simulink model "model"  (R2024a)
settings: Solver=FixedStepDiscrete  StartTime=0.0  StopTime=Tend  FixedStep=Ts  RelTol=1e-3
PreLoadFcn:
  | release_bus_types;
InitFcn:
  | release_initialize(p1,p2,p3,p4);
StartFcn:
  | % MG_4bus_ini;
values from neighbouring files (symbols this model uses):
  dPQload_max = 100*S_b    (= 100000)    [ini.m]
  f_b = 60    [ini.m]
  I_b = S_b/(sqrt(3)*V_b)    [ini.m]
  S_b = 1e3    (= 1000)    [ini.m]
  V_b = 230    [ini.m]
  V_m = sqrt(2/3)*V_b    [ini.m]
  Vdc_n = 3*V_m    [ini.m]
undefined symbols (not defined in the file or in its folder): DynLoad_Ps, DynLoad_Qs, p1, p2, p3, p4, Ts
libraries: lib_IBR x24, spsabctodq0Lib x20, spsSeriesRLCBranchLib x18, spsThreePhaseVIMeasurementLib x8, spsThreePhaseSeriesRLCBranchLib x8, spsThreePhaseSeriesRLCLoadLib x4, spsDCVoltageSourceLib x4, spsUniversalBridgeLib x4, spsControlledVoltageSourceLib x3, spsPowerdq0InstantaneousLib x2, spsdq0toabcLib x2, spsThreePhaseDynamicLoadLib x1
settings Model: SimulationMode=accelerator  Creator=mdu9  LastModifiedBy=mdu9
settings OptimizationCC: DefaultParameterBehavior=Inlined  EnhancedBackFolding=on  PassReuseOutputArgsThreshold=0  AccelVerboseBuild=on  OptimizeBlockOrder=speed  DifferentSizesBufferReuse=on  OptimizationCustomize=off
settings DebuggingCC: SaveWithDisabledLinksMsg=none  SaveWithParameterizedLinksMsg=error  ParameterTunabilityLossMsg=error
settings SFSimCC: MATLABDynamicMemAlloc=off
settings RTWCC: GPUComputeCapability=3.5
settings CodeAppCC: ForceParamTrailComments=on  OperatorAnnotations=on

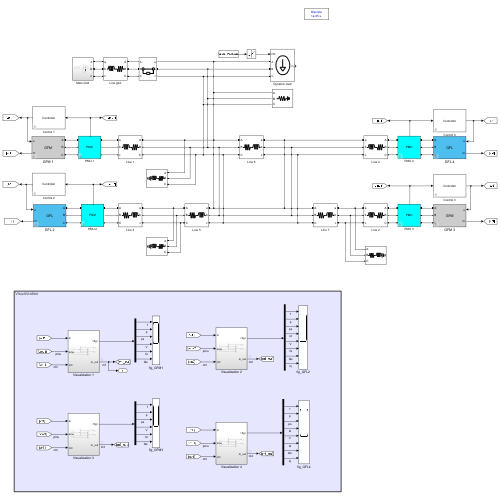
[thumbnail: Simulink's stored preview of the top-level diagram]
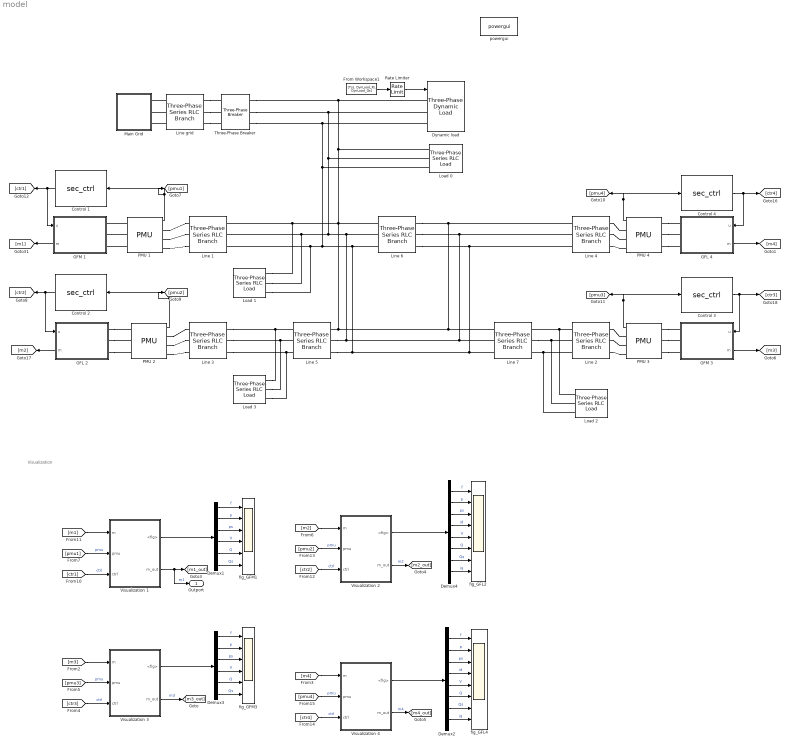
== system model ==
  note: Visualization
  " Load 1" : spsThreePhaseSeriesRLCLoadLib/Three-Phase Series RLC Load  LConnTagsString=A|B|C  Configuration=Y (grounded)  NominalVoltage=V_b  Vabc=[1e3 1e3 1e3]  Vabcp=[1e3 1e3 1e3]  NominalFrequency=f_b  UnbalancedPower=off  ActivePower=Pload1  InductivePower=Qload1  CapacitivePower=0  Pabc=[10e3 9e3 11e3]  QLabc=[100 90 110]  QCabc=[100 90 110]  Pabcp=[10e3 9e3 11e3]  QLabcp=[100 90 110]  QCabcp=[100 90 110]  Measurements=None  LoadType=constant PQ
  " Load 2" : spsThreePhaseSeriesRLCLoadLib/Three-Phase Series RLC Load  LConnTagsString=A|B|C  Configuration=Y (grounded)  NominalVoltage=V_b  Vabc=[1e3 1e3 1e3]  Vabcp=[1e3 1e3 1e3]  NominalFrequency=f_b  UnbalancedPower=off  ActivePower=Pload1  InductivePower=Qload1  CapacitivePower=0  Pabc=[10e3 9e3 11e3]  QLabc=[100 90 110]  QCabc=[100 90 110]  Pabcp=[10e3 9e3 11e3]  QLabcp=[100 90 110]  QCabcp=[100 90 110]  Measurements=None  LoadType=constant PQ
  " Load 3" : spsThreePhaseSeriesRLCLoadLib/Three-Phase Series RLC Load  LConnTagsString=A|B|C  Configuration=Y (grounded)  NominalVoltage=V_b  Vabc=[1e3 1e3 1e3]  Vabcp=[1e3 1e3 1e3]  NominalFrequency=f_b  UnbalancedPower=off  ActivePower=Pload1  InductivePower=Qload1  CapacitivePower=0  Pabc=[10e3 9e3 11e3]  QLabc=[100 90 110]  QCabc=[100 90 110]  Pabcp=[10e3 9e3 11e3]  QLabcp=[100 90 110]  QCabcp=[100 90 110]  Measurements=None  LoadType=constant PQ
  Control 1 : lib_IBR/sec_ctrl  pIBR=p1
  Control 2 : lib_IBR/sec_ctrl  pIBR=p2
  Control 3 : lib_IBR/sec_ctrl  pIBR=p3
  Control 4 : lib_IBR/sec_ctrl  pIBR=p4
  Demux1 : Demux  Outputs=[2,1,1,2,1,1]
  Demux2 : Demux  Outputs=[1, 1, 1, 2, 1, 1, 1, 2]
  Demux3 : Demux  Outputs=[2,1,1,2,1,1]
  Demux4 : Demux  Outputs=[1, 1, 1, 2, 1, 1, 1, 2]
  Dynamic load : spsThreePhaseDynamicLoadLib/Three-Phase Dynamic Load  NominalVoltage=[ V_b f_b ]  ActiveReactivePowers=[DynLoad_Ps(1) DynLoad_Qs(1)]  PositiveSequence=[0.994 -11.8]  ExternalControl=on  NpNq=[1.3 2]  TimeConstants="[0  0  0  0]"  MinimumVoltage=0.7  Tfilter=Ts  LoadFlowParameters=[4,0,0,0,0]
      settings: LibrarySourceBlock=|
      | sps_lib/Passives/Three-Phase
      | Dynamic Load
  From Workspace1 : FromWorkspace  VariableName=[Tss, DynLoad_Ps, DynLoad_Qs]  SampleTime=Ts
  GFL 2 : Subsystem  Tag=VSI  Description=VSI  mask{pIBR=p2}
      mask prompts: pIBR "IBR parameters"
      settings: PortSchema="{\"entries\":[{\"content\":{\"sides\":[{\"content\":{\"connectorIds\":[\"In1\",\"Out1\"]},\"type\":\"ConnectorPlacement.EquallySpacedRectSide\",\"uuid\":\"7a695335-592e-4119-9ab1-0e8bf6eac77e\"},{\"content\":{\"connectorIds\":[\"RConn1\",\"RConn2\",\"RConn3\"],\"side\":\"RIGHT\"},\"type\":\"ConnectorPlacement.EquallySpacedRectSide\",\"uuid\":\"49a3a23c-5004-48bd-b13d-54549b783a30\"},{\"content\":{\"side\":\"TOP\"},\"type\":\"ConnectorPlacement.EquallySpacedRectSide\",\"uuid\":\"db95583c-7fb3-4e7b-a0da-760f8ba1f545\"}]},\"type\":\"ConnectorPlacement.EquallySpacedConnector\",\"uuid\":\"af105942-44d0-4ac1-b36b-d1c23a009ef5\"}],\"packageUris\":[\"http://schema.mathworks.com/mf0/Connector/R2020b\"],\"version\":\"1.0\"}"
      mask Display: disp('GFL')
  GFL 4 : Subsystem  Tag=VSI  Description=VSI  mask{pIBR=p4}
      mask prompts: pIBR "IBR parameters"
      settings: PortSchema="{\"entries\":[{\"content\":{\"sides\":[{\"content\":{\"connectorIds\":[\"In1\",\"Out1\"]},\"type\":\"ConnectorPlacement.EquallySpacedRectSide\",\"uuid\":\"7a695335-592e-4119-9ab1-0e8bf6eac77e\"},{\"content\":{\"connectorIds\":[\"RConn1\",\"RConn2\",\"RConn3\"],\"side\":\"RIGHT\"},\"type\":\"ConnectorPlacement.EquallySpacedRectSide\",\"uuid\":\"49a3a23c-5004-48bd-b13d-54549b783a30\"},{\"content\":{\"side\":\"TOP\"},\"type\":\"ConnectorPlacement.EquallySpacedRectSide\",\"uuid\":\"db95583c-7fb3-4e7b-a0da-760f8ba1f545\"}]},\"type\":\"ConnectorPlacement.EquallySpacedConnector\",\"uuid\":\"af105942-44d0-4ac1-b36b-d1c23a009ef5\"}],\"packageUris\":[\"http://schema.mathworks.com/mf0/Connector/R2020b\"],\"version\":\"1.0\"}"
      mask Display: disp('GFL')
  GFM 1 : Subsystem  mask{pIBR=p1}
      mask prompts: pIBR "IBR parameters"
      settings: PortSchema="{\"entries\":[{\"content\":{\"sides\":[{\"content\":{\"connectorIds\":[\"In1\",\"Out1\"]},\"type\":\"ConnectorPlacement.EquallySpacedRectSide\",\"uuid\":\"7a695335-592e-4119-9ab1-0e8bf6eac77e\"},{\"content\":{\"connectorIds\":[\"RConn1\",\"RConn2\",\"RConn3\"],\"side\":\"RIGHT\"},\"type\":\"ConnectorPlacement.EquallySpacedRectSide\",\"uuid\":\"49a3a23c-5004-48bd-b13d-54549b783a30\"},{\"content\":{\"side\":\"TOP\"},\"type\":\"ConnectorPlacement.EquallySpacedRectSide\",\"uuid\":\"db95583c-7fb3-4e7b-a0da-760f8ba1f545\"}]},\"type\":\"ConnectorPlacement.EquallySpacedConnector\",\"uuid\":\"af105942-44d0-4ac1-b36b-d1c23a009ef5\"}],\"packageUris\":[\"http://schema.mathworks.com/mf0/Connector/R2020b\"],\"version\":\"1.0\"}"
      mask Display: disp('GFM')
  GFM 3 : Subsystem  mask{pIBR=p3}
      mask prompts: pIBR "IBR parameters"
      settings: PortSchema="{\"entries\":[{\"content\":{\"sides\":[{\"content\":{\"connectorIds\":[\"In1\",\"Out1\"]},\"type\":\"ConnectorPlacement.EquallySpacedRectSide\",\"uuid\":\"7a695335-592e-4119-9ab1-0e8bf6eac77e\"},{\"content\":{\"connectorIds\":[\"RConn1\",\"RConn2\",\"RConn3\"],\"side\":\"RIGHT\"},\"type\":\"ConnectorPlacement.EquallySpacedRectSide\",\"uuid\":\"49a3a23c-5004-48bd-b13d-54549b783a30\"},{\"content\":{\"side\":\"TOP\"},\"type\":\"ConnectorPlacement.EquallySpacedRectSide\",\"uuid\":\"db95583c-7fb3-4e7b-a0da-760f8ba1f545\"}]},\"type\":\"ConnectorPlacement.EquallySpacedConnector\",\"uuid\":\"af105942-44d0-4ac1-b36b-d1c23a009ef5\"}],\"packageUris\":[\"http://schema.mathworks.com/mf0/Connector/R2020b\"],\"version\":\"1.0\"}"
      mask Display: disp('GFM')
  Line {1..6} (6 alike) : spsThreePhaseSeriesRLCBranchLib/Three-Phase Series RLC Branch  LConnTagsString=A|B|C  RConnTagsString=A|B|C  BranchType=RL  Resistance=0.2  Inductance=0.0002  Capacitance=1e-6  Measurements=None
  Line 7 : spsThreePhaseSeriesRLCBranchLib/Three-Phase Series RLC Branch  LConnTagsString=A|B|C  RConnTagsString=A|B|C  BranchType=RL  Resistance=6  Inductance=0.006  Capacitance=1e-6  Measurements=None
  Line grid : spsThreePhaseSeriesRLCBranchLib/Three-Phase Series RLC Branch  LConnTagsString=A|B|C  RConnTagsString=A|B|C  BranchType=RL  Resistance=2  Inductance=0.00022  Capacitance=1e-6  Measurements=None
  Load 0 : spsThreePhaseSeriesRLCLoadLib/Three-Phase Series RLC Load  LConnTagsString=A|B|C  Configuration=Y (grounded)  NominalVoltage=V_b  Vabc=[1e3 1e3 1e3]  Vabcp=[1e3 1e3 1e3]  NominalFrequency=f_b  UnbalancedPower=off  ActivePower=Pload0  InductivePower=0  CapacitivePower=0  Pabc=[10e3 9e3 11e3]  QLabc=[100 90 110]  QCabc=[100 90 110]  Pabcp=[10e3 9e3 11e3]  QLabcp=[100 90 110]  QCabcp=[100 90 110]  Measurements=None  LoadType=constant PQ
  Main Grid : Subsystem
  PMU 1 : lib_IBR/PMU  pIBR=p1
  PMU 2 : lib_IBR/PMU  pIBR=p2
  PMU 3 : lib_IBR/PMU  pIBR=p3
  PMU 4 : lib_IBR/PMU  pIBR=p4
  Rate Limiter : RateLimiter  RisingSlewLimit=dPQload_max  FallingSlewLimit=-dPQload_max  SampleTimeMode=inherited
  Three-Phase Breaker : spsThreePhaseBreakerLib/Three-Phase Breaker  InitialState=closed  SwitchA=on  SwitchB=on  SwitchC=on  SwitchTimes=T_island  External=off  BreakerResistance=0.01  SnubberResistance=1e6  SnubberCapacitance=inf  Measurements=None
  Visualization 1 : Subsystem
  Visualization 2 : Subsystem
  Visualization 3 : Subsystem
  Visualization 4 : Subsystem
  fig_GFL2 : Scope  NumInputPorts=8
  fig_GFL4 : Scope  NumInputPorts=8
  fig_GFM1 : Scope  NumInputPorts=6
  fig_GFM3 : Scope  NumInputPorts=6
  powergui : spspowerguiLib/powergui  Priority=1  SimulationMode=Discrete  SampleTime=Ts  frequency=60  Iterations=50  frequencyindice=0  Pbase=100e6  ErrMax=1e-4  UnitsV=kV  UnitsW=MW  buscounter=0  FunctionMessages=off  echomessages=off  EnableUseOfTLC=off  CurrentSourceSwitches=off  DisableSnubberDevices=off  DisableRonSwitches=off  DisableVfSwitches=off  DisplayEquations=off  AutomaticDiscreteSolvers=off  SolverType=Tustin/Backward Euler (TBE)  Interpol=off  ExternalGateDelay=off  methode=off  Ts=100  x0status=blocks  SPID=on  SwTol=0  HookPort=off  NonlinearTolerance=1e-4  nMaxIteration=100  ContinueOnMaxIteration=off  RestoreLinks=warning  ResistiveCurrentMeasurement=off  Frange=[0:2:500]  Ylog=off  Xlog=on  ShowGrid=off  save=off  variable=ZData  structure=0  ZoomFFT=off  StartTime=0.0  cycles=1  DisplayStyle=1  fundamental=60  FreqAxis=off  MaxFrequency=1000  frequencyindicesteady=1  RmsSteady=1  display=off
  Outport : Outport
  wires:
  GFM 1/1(m) -> [m1]
  From Workspace1/1 -> Rate Limiter/1
  GFM 3/1(m) -> [m3]
  Demux3/4 -> fig_GFM3/4  "V"
  Demux3/1 -> fig_GFM3/1  "f"
  Demux3/6 -> fig_GFM3/6  "Qs"
  Demux3/5 -> fig_GFM3/5  "Q"
  Demux3/3 -> fig_GFM3/3  "ps"
  Demux3/2 -> fig_GFM3/2  "p"
  GFL 2/1(m) -> [m2]
  Demux4/1 -> fig_GFL2/1  "f"
  Demux4/2 -> fig_GFL2/2  "p"
  Demux4/3 -> fig_GFL2/3  "ps"
  Demux4/4 -> fig_GFL2/4  "id"
  Demux4/5 -> fig_GFL2/5  "V"
  Demux4/6 -> fig_GFL2/6  "Q"
  Demux4/7 -> fig_GFL2/7  "Qs"
  Demux4/8 -> fig_GFL2/8  "iq"
  GFL 4/1(m) -> [m4]
  Demux2/8 -> fig_GFL4/8  "iq"
  Demux2/7 -> fig_GFL4/7  "Qs"
  Demux2/6 -> fig_GFL4/6  "Q"
  Demux2/5 -> fig_GFL4/5  "V"
  Demux2/4 -> fig_GFL4/4  "id"
  Demux2/3 -> fig_GFL4/3  "ps"
  Demux2/2 -> fig_GFL4/2  "p"
  Demux2/1 -> fig_GFL4/1  "f"
  Demux1/1 -> fig_GFM1/1  "f"
  Demux1/2 -> fig_GFM1/2  "p"
  Demux1/6 -> fig_GFM1/6  "Qs"
  Demux1/5 -> fig_GFM1/5  "Q"
  Demux1/4 -> fig_GFM1/4  "V"
  Demux1/3 -> fig_GFM1/3  "ps"
  Rate Limiter/1 -> Dynamic load/1
  PMU 1/1 -> [pmu1], Control 1/1
  PMU 4/1 -> [pmu4], Control 4/1
  PMU 3/1 -> [pmu3], Control 3/1
  PMU 2/1 -> [pmu2], Control 2/1
  Visualization 1/2(m_out) -> [m1_out], Outport/1  "m1"
  [m1] -> Visualization 1/1(m)
  [pmu1] -> Visualization 1/2(pmu)  "pmu"
  [ctr1] -> Visualization 1/3(ctrl)  "ctrl"
  Visualization 1/1(<fig>) -> Demux1/1
  [m2] -> Visualization 2/1(m)
  [ctr2] -> Visualization 2/3(ctrl)  "ctrl"
  [pmu2] -> Visualization 2/2(pmu)  "pmu"
  Visualization 2/2(m_out) -> [m2_out]  "m2"
  Visualization 2/1(<fig>) -> Demux4/1
  [m3] -> Visualization 3/1(m)
  [ctr3] -> Visualization 3/3(ctrl)  "ctrl"
  [pmu3] -> Visualization 3/2(pmu)  "pmu"
  Visualization 3/2(m_out) -> [m3_out]  "m3"
  Visualization 3/1(<fig>) -> Demux3/1
  [ctr4] -> Visualization 4/3(ctrl)  "ctrl"
  [pmu4] -> Visualization 4/2(pmu)  "pmu"
  [m4] -> Visualization 4/1(m)
  Visualization 4/2(m_out) -> [m4_out]  "m4"
  Visualization 4/1(<fig>) -> Demux2/1
  Control 1/1 -> GFM 1/1(u), [ctr1]
  Control 2/1 -> [ctr2], GFL 2/1(u)
  Control 3/1 -> [ctr3], GFM 3/1(u)
  Control 4/1 -> [ctr4], GFL 4/1(u)
  connections:
  Line grid/LConn2 -- Three-Phase Breaker/LConn2
  Line grid/LConn1 -- Three-Phase Breaker/LConn1
  Line grid/LConn3 -- Three-Phase Breaker/LConn3
  Line grid/RConn3 -- Main Grid/RConn3
  Line grid/RConn2 -- Main Grid/RConn2
  Line grid/RConn1 -- Main Grid/RConn1
  Line 4/RConn1 -- Line 6/RConn1 -- Three-Phase Breaker/RConn1 -- Dynamic load/LConn1 -- Load 0/LConn1 -- Line 6/LConn1 -- " Load 1"/LConn1 -- Line 1/LConn1 -- Line 5/RConn1 -- Line 7/LConn1
  " Load 2"/LConn2 -- Line 7/RConn2 -- Line 2/RConn2
  " Load 1"/LConn2 -- Three-Phase Breaker/RConn2 -- Dynamic load/LConn2 -- Load 0/LConn2 -- Line 6/LConn2 -- Line 7/LConn2 -- Line 6/RConn2 -- Line 4/RConn2 -- Line 5/RConn2 -- Line 1/LConn2
  " Load 1"/LConn3 -- Three-Phase Breaker/RConn3 -- Dynamic load/LConn3 -- Load 0/LConn3 -- Line 6/LConn3 -- Line 7/LConn3 -- Line 4/RConn3 -- Line 6/RConn3 -- Line 5/RConn3 -- Line 1/LConn3
  Line 3/RConn2 -- Line 5/LConn2 -- " Load 3"/LConn2
  Line 3/RConn1 -- Line 5/LConn1 -- " Load 3"/LConn1
  Line 3/RConn3 -- Line 5/LConn3 -- " Load 3"/LConn3
  " Load 2"/LConn1 -- Line 7/RConn1 -- Line 2/RConn1
  " Load 2"/LConn3 -- Line 7/RConn3 -- Line 2/RConn3
  PMU 1/LConn1 -- GFM 1/RConn1
  PMU 1/LConn2 -- GFM 1/RConn2
  PMU 1/LConn3 -- GFM 1/RConn3
  PMU 1/RConn1 -- Line 1/RConn1
  PMU 1/RConn2 -- Line 1/RConn2
  PMU 1/RConn3 -- Line 1/RConn3
  GFL 2/RConn1 -- PMU 2/LConn1
  GFL 2/RConn2 -- PMU 2/LConn2
  GFL 2/RConn3 -- PMU 2/LConn3
  PMU 2/RConn1 -- Line 3/LConn1
  PMU 2/RConn2 -- Line 3/LConn2
  PMU 4/RConn1 -- Line 4/LConn1
  PMU 4/RConn2 -- Line 4/LConn2
  PMU 4/RConn3 -- Line 4/LConn3
  PMU 4/LConn1 -- GFL 4/RConn1
  PMU 4/LConn2 -- GFL 4/RConn2
  PMU 4/LConn3 -- GFL 4/RConn3
  PMU 3/LConn2 -- GFM 3/RConn2
  PMU 3/LConn1 -- GFM 3/RConn1
  PMU 3/LConn3 -- GFM 3/RConn3
  PMU 3/RConn2 -- Line 2/LConn2
  PMU 3/RConn1 -- Line 2/LConn1
  PMU 3/RConn3 -- Line 2/LConn3
  PMU 2/RConn3 -- Line 3/LConn3

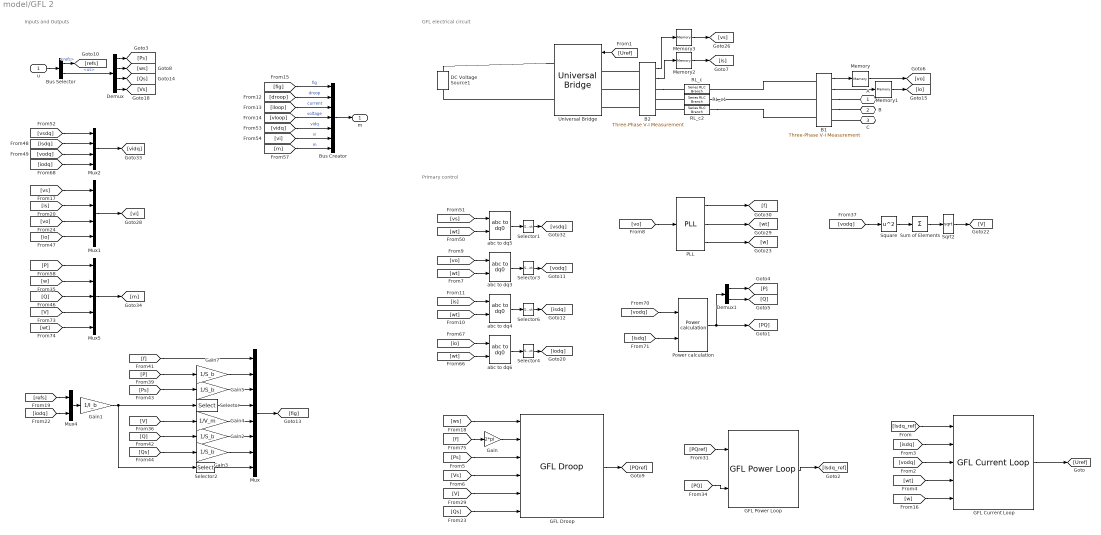
== system model/GFL 2 ==
  note: Inputs and Outputs
  note: GFL electrical circuit
  note: Primary control
  u : Inport
  B1 : spsThreePhaseVIMeasurementLib/Three-Phase V-I Measurement  VoltageMeasurement=phase-to-ground  SetLabelV=off  LabelV=v  Vpu=off  VpuLL=off  CurrentMeasurement=yes  SetLabelI=off  LabelI=i  Ipu=off  Pbase=Pbase  Vbase=Vbase  OutputType=Magnitude  PhasorSimulation=off  PSBequivalent=0
  B2 : spsThreePhaseVIMeasurementLib/Three-Phase V-I Measurement  VoltageMeasurement=phase-to-ground  SetLabelV=off  LabelV=v  Vpu=off  VpuLL=off  CurrentMeasurement=yes  SetLabelI=off  LabelI=i  Ipu=off  Pbase=Pbase  Vbase=Vbase  OutputType=Magnitude  PhasorSimulation=off  PSBequivalent=0
  Bus Creator : BusCreator  Inputs=7
  Bus Selector : BusSelector  OutputSignals=refs,us
  DC Voltage Source1 : spsDCVoltageSourceLib/DC Voltage Source  Amplitude=Vdc_n  Measurements=None
  Demux : Demux
  Demux1 : Demux  Outputs=2
  GFL Current Loop : lib_IBR/GFL Current Loop  SystemSampleTime=-1  VariantActivationTime=update diagram  AllowFlexibleInterface=on  Latency=0  AutoFrameSizeCalculation=off
  "GFL Droop " : lib_IBR/GFL Droop   SystemSampleTime=-1  VariantActivationTime=update diagram  AllowFlexibleInterface=on  Latency=0  AutoFrameSizeCalculation=off
  GFL Power Loop : lib_IBR/GFL Power Loop  SystemSampleTime=-1  VariantActivationTime=update diagram  AllowFlexibleInterface=on  Latency=0  AutoFrameSizeCalculation=off
  Gain : Gain  Gain=2*pi
  Gain1 : Gain  Gain=1/I_b
  Gain{2..3,5,7} (4 alike) : Gain  Gain=1/S_b
  Gain4 : Gain  Gain=1/V_m
  Memory{,1..3} (4 alike) : Memory
  Mux : Mux  Inputs=8
  Mux1 : Mux
  Mux2 : Mux
  Mux4 : Mux  Inputs=2
  Mux5 : Mux  Inputs=5
  PLL : lib_IBR/PLL  Frng=pIBR.pll.frng  Par_Init=[0 f_b]  ParK=pIBR.pll.Kpi  TcD=1e-4  MaxRateChangeFreq=pIBR.pll.dfrng  FilterCutOffFreq=pIBR.pll.fc  Ts=Ts  AGC=0
  Power calculation : lib_IBR/Power calculation  SystemSampleTime=-1  VariantActivationTime=update diagram  AllowFlexibleInterface=on  Latency=0  AutoFrameSizeCalculation=off
  RL_c : spsSeriesRLCBranchLib/Series RLC Branch  LConnTagsString=__new0  RConnTagsString=__new0  BranchType=RL  Resistance=pIBR.RLC(1)  Inductance=pIBR.RLC(2)  SetiL0=off  InitialCurrent=0  Capacitance=1e-6  Setx0=off  InitialVoltage=0  Measurements=None
  RL_c1 : spsSeriesRLCBranchLib/Series RLC Branch  LConnTagsString=__new0  RConnTagsString=__new0  BranchType=RL  Resistance=pIBR.RLC(1)  Inductance=pIBR.RLC(2)  SetiL0=off  InitialCurrent=0  Capacitance=1e-6  Setx0=off  InitialVoltage=0  Measurements=None
  RL_c2 : spsSeriesRLCBranchLib/Series RLC Branch  LConnTagsString=__new0  RConnTagsString=__new0  BranchType=RL  Resistance=pIBR.RLC(1)  Inductance=pIBR.RLC(2)  SetiL0=off  InitialCurrent=0  Capacitance=1e-6  Setx0=off  InitialVoltage=0  Measurements=None
  Selector : Selector  InputPortWidth=4  IndexOptions=Index vector (dialog)  Indices=[1 3]  OutputSizes=1
  Selector{1,3..4,6} (4 alike) : Selector  InputPortWidth=3  IndexOptions=Index vector (dialog)  Indices=[1 2]  OutputSizes=1
  Selector2 : Selector  InputPortWidth=4  IndexOptions=Index vector (dialog)  Indices=[2 4]  OutputSizes=1
  Sqrt2 : Sqrt
  Square : Math  Operator=square
  Sum of Elements : Sum  Inputs=+
  Universal Bridge : spsUniversalBridgeLib/Universal Bridge  Arms=3  SnubberResistance=1e5  SnubberCapacitance=inf  Device=Average-model based VSC  Ron=1e-3  Lon=0  ForwardVoltages="[  0  0  ]"  ForwardVoltage=0  GTOparameters=[ 10e-6 , 20e-6 ]  IGBTparameters=[ 1e-6 , 2e-6 ]  Measurements=None  Measurements_2=None  converterType=Rectifier
  abc to dq{3..6} (4 alike) : spsabctodq0Lib/abc to dq0  Alignment=90 degrees behind phase A axis
  A : PMIOPort  Side=Right
  B : PMIOPort  Port=2  Side=Right
  C : PMIOPort  Port=3  Side=Right
  m : Outport  VectorParamsAs1DForOutWhenUnconnected=off
  wires:
  [refs] -> Mux4/1
  Demux/4 -> [Vs]
  Demux/3 -> [Qs]
  Demux/2 -> [ws]
  Demux/1 -> [Ps]
  [wt] -> Mux5/5
  [V] -> Mux5/4
  [Q] -> Mux5/3
  [f] -> Gain/1
  Mux5/1 -> [m]
  [P] -> Mux5/1
  [w] -> Mux5/2
  [Qs] -> Gain3/1
  [Ps] -> Gain5/1
  [vodq] -> GFL Current Loop/3
  [isdq] -> GFL Current Loop/2
  [Isdq_ref] -> GFL Current Loop/1
  GFL Current Loop/1 -> [Uref]
  B1/1 -> Memory/1
  [wt] -> abc to dq3/2
  Selector3/1 -> [vodq]
  [vo] -> abc to dq3/1
  abc to dq3/1 -> Selector3/1
  [wt] -> abc to dq4/2
  abc to dq4/1 -> Selector6/1
  Selector6/1 -> [isdq]
  [wt] -> GFL Current Loop/4
  B2/2 -> Memory2/1
  B1/2 -> Memory1/1
  "GFL Droop "/1 -> [PQref]
  GFL Power Loop/1 -> [Isdq_ref]
  u/1 -> Bus Selector/1
  [Ps] -> "GFL Droop "/3
  [Vs] -> "GFL Droop "/4
  [ws] -> "GFL Droop "/1
  [Qs] -> "GFL Droop "/6
  Gain/1 -> "GFL Droop "/2
  [V] -> "GFL Droop "/5
  [PQref] -> GFL Power Loop/1
  [PQ] -> GFL Power Loop/2
  Mux/1 -> [fig]
  [f] -> Mux/1
  [P] -> Gain7/1
  [V] -> Gain4/1
  [vodq] -> Square/1
  Sum of Elements/1 -> Sqrt2/1
  [Q] -> Gain2/1
  Memory2/1 -> [is]
  Memory/1 -> [vo]
  Memory1/1 -> [io]
  [is] -> abc to dq4/1
  Memory3/1 -> [vs]
  B2/1 -> Memory3/1
  [vo] -> PLL/1
  PLL/2 -> [wt]
  PLL/1 -> [f]
  Bus Creator/1 -> m/1
  [droop] -> Bus Creator/2  "droop"
  [iloop] -> Bus Creator/3  "current"
  [vloop] -> Bus Creator/4  "voltage"
  [fig] -> Bus Creator/1  "fig"
  PLL/3 -> [w]
  [w] -> GFL Current Loop/5
  [vs] -> Mux1/1
  [is] -> Mux1/2
  [vo] -> Mux1/3
  [io] -> Mux1/4
  Mux1/1 -> [vi]
  [vs] -> abc to dq5/1
  Selector1/1 -> [vsdq]
  [wt] -> abc to dq5/2
  abc to dq5/1 -> Selector1/1
  [vsdq] -> Mux2/1
  [isdq] -> Mux2/2
  [vodq] -> Mux2/3
  Mux2/1 -> [vidq]
  [vidq] -> Bus Creator/5  "vidq"
  [vi] -> Bus Creator/6  "vi"
  [m] -> Bus Creator/7  "m"
  [io] -> abc to dq6/1
  abc to dq6/1 -> Selector4/1
  [wt] -> abc to dq6/2
  Selector4/1 -> [iodq]
  [iodq] -> Mux2/4
  Square/1 -> Sum of Elements/1
  [isdq] -> Power calculation/2
  [vodq] -> Power calculation/1
  [Uref] -> Universal Bridge/1
  Power calculation/1 -> Demux1/1, [PQ]
  Demux1/1 -> [P]
  Demux1/2 -> [Q]
  Sqrt2/1 -> [V]
  Gain7/1 -> Mux/2
  Gain5/1 -> Mux/3
  Bus Selector/1 -> [refs]  "<refs>"
  [iodq] -> Mux4/2
  Mux4/1 -> Gain1/1
  Selector/1 -> Mux/4
  Gain4/1 -> Mux/5
  Gain2/1 -> Mux/6
  Gain3/1 -> Mux/7
  Selector2/1 -> Mux/8
  Gain1/1 -> Selector2/1, Selector/1
  Bus Selector/2 -> Demux/1  "<us>"
  connections:
  Universal Bridge/RConn2 -- DC Voltage Source1/LConn1
  Universal Bridge/RConn1 -- DC Voltage Source1/RConn1
  RL_c2/LConn1 -- B1/LConn3
  B2/LConn2 -- Universal Bridge/LConn2
  B2/LConn1 -- Universal Bridge/LConn1
  B2/LConn3 -- Universal Bridge/LConn3
  C/RConn1 -- B1/RConn3
  B1/RConn2 -- B/RConn1
  B1/RConn1 -- A/RConn1
  B1/LConn1 -- RL_c/LConn1
  RL_c1/LConn1 -- B1/LConn2
  RL_c2/RConn1 -- B2/RConn3
  RL_c1/RConn1 -- B2/RConn2
  B2/RConn1 -- RL_c/RConn1

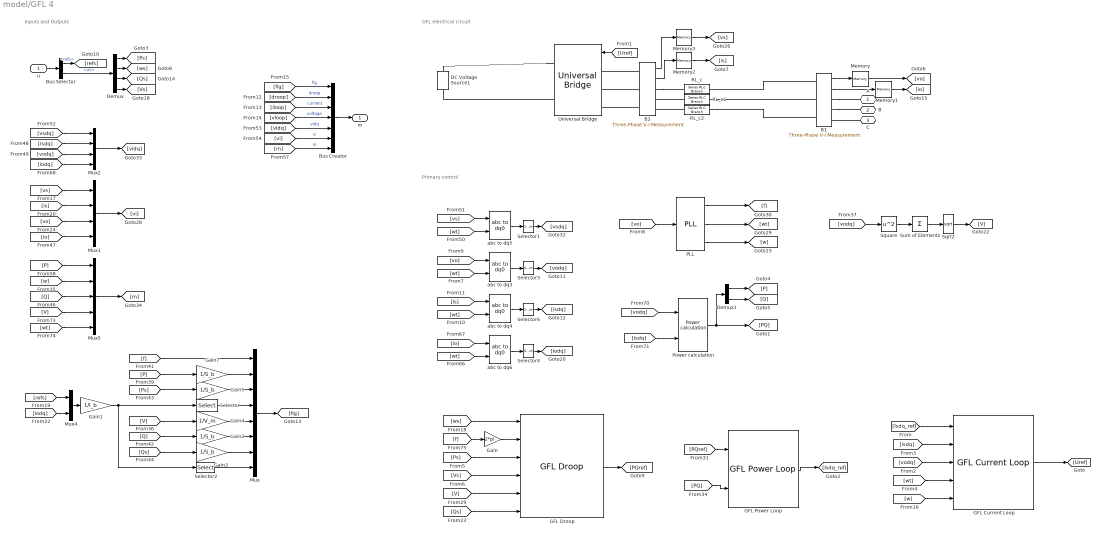
== system model/GFL 4 ==
  note: Inputs and Outputs
  note: GFL electrical circuit
  note: Primary control
  u : Inport
  B1 : spsThreePhaseVIMeasurementLib/Three-Phase V-I Measurement  VoltageMeasurement=phase-to-ground  SetLabelV=off  LabelV=v  Vpu=off  VpuLL=off  CurrentMeasurement=yes  SetLabelI=off  LabelI=i  Ipu=off  Pbase=Pbase  Vbase=Vbase  OutputType=Magnitude  PhasorSimulation=off  PSBequivalent=0
  B2 : spsThreePhaseVIMeasurementLib/Three-Phase V-I Measurement  VoltageMeasurement=phase-to-ground  SetLabelV=off  LabelV=v  Vpu=off  VpuLL=off  CurrentMeasurement=yes  SetLabelI=off  LabelI=i  Ipu=off  Pbase=Pbase  Vbase=Vbase  OutputType=Magnitude  PhasorSimulation=off  PSBequivalent=0
  Bus Creator : BusCreator  Inputs=7
  Bus Selector : BusSelector  OutputSignals=refs,us
  DC Voltage Source1 : spsDCVoltageSourceLib/DC Voltage Source  Amplitude=Vdc_n  Measurements=None
  Demux : Demux
  Demux1 : Demux  Outputs=2
  GFL Current Loop : lib_IBR/GFL Current Loop  SystemSampleTime=-1  VariantActivationTime=update diagram  AllowFlexibleInterface=on  Latency=0  AutoFrameSizeCalculation=off
  "GFL Droop " : lib_IBR/GFL Droop   SystemSampleTime=-1  VariantActivationTime=update diagram  AllowFlexibleInterface=on  Latency=0  AutoFrameSizeCalculation=off
  GFL Power Loop : lib_IBR/GFL Power Loop  SystemSampleTime=-1  VariantActivationTime=update diagram  AllowFlexibleInterface=on  Latency=0  AutoFrameSizeCalculation=off
  Gain : Gain  Gain=2*pi
  Gain1 : Gain  Gain=1/I_b
  Gain{2..3,5,7} (4 alike) : Gain  Gain=1/S_b
  Gain4 : Gain  Gain=1/V_m
  Memory{,1..3} (4 alike) : Memory
  Mux : Mux  Inputs=8
  Mux1 : Mux
  Mux2 : Mux
  Mux4 : Mux  Inputs=2
  Mux5 : Mux  Inputs=5
  PLL : lib_IBR/PLL  Frng=pIBR.pll.frng  Par_Init=[0 f_b]  ParK=pIBR.pll.Kpi  TcD=1e-4  MaxRateChangeFreq=pIBR.pll.dfrng  FilterCutOffFreq=pIBR.pll.fc  Ts=Ts  AGC=0
  Power calculation : lib_IBR/Power calculation  SystemSampleTime=-1  VariantActivationTime=update diagram  AllowFlexibleInterface=on  Latency=0  AutoFrameSizeCalculation=off
  RL_c : spsSeriesRLCBranchLib/Series RLC Branch  LConnTagsString=__new0  RConnTagsString=__new0  BranchType=RL  Resistance=pIBR.RLC(1)  Inductance=pIBR.RLC(2)  SetiL0=off  InitialCurrent=0  Capacitance=1e-6  Setx0=off  InitialVoltage=0  Measurements=None
  RL_c1 : spsSeriesRLCBranchLib/Series RLC Branch  LConnTagsString=__new0  RConnTagsString=__new0  BranchType=RL  Resistance=pIBR.RLC(1)  Inductance=pIBR.RLC(2)  SetiL0=off  InitialCurrent=0  Capacitance=1e-6  Setx0=off  InitialVoltage=0  Measurements=None
  RL_c2 : spsSeriesRLCBranchLib/Series RLC Branch  LConnTagsString=__new0  RConnTagsString=__new0  BranchType=RL  Resistance=pIBR.RLC(1)  Inductance=pIBR.RLC(2)  SetiL0=off  InitialCurrent=0  Capacitance=1e-6  Setx0=off  InitialVoltage=0  Measurements=None
  Selector : Selector  InputPortWidth=4  IndexOptions=Index vector (dialog)  Indices=[1 3]  OutputSizes=1
  Selector{1,3..4,6} (4 alike) : Selector  InputPortWidth=3  IndexOptions=Index vector (dialog)  Indices=[1 2]  OutputSizes=1
  Selector2 : Selector  InputPortWidth=4  IndexOptions=Index vector (dialog)  Indices=[2 4]  OutputSizes=1
  Sqrt2 : Sqrt
  Square : Math  Operator=square
  Sum of Elements : Sum  Inputs=+
  Universal Bridge : spsUniversalBridgeLib/Universal Bridge  Arms=3  SnubberResistance=1e5  SnubberCapacitance=inf  Device=Average-model based VSC  Ron=1e-3  Lon=0  ForwardVoltages="[  0  0  ]"  ForwardVoltage=0  GTOparameters=[ 10e-6 , 20e-6 ]  IGBTparameters=[ 1e-6 , 2e-6 ]  Measurements=None  Measurements_2=None  converterType=Rectifier
  abc to dq{3..6} (4 alike) : spsabctodq0Lib/abc to dq0  Alignment=90 degrees behind phase A axis
  A : PMIOPort  Side=Right
  B : PMIOPort  Port=2  Side=Right
  C : PMIOPort  Port=3  Side=Right
  m : Outport  VectorParamsAs1DForOutWhenUnconnected=off
  wires:
  [refs] -> Mux4/1
  Demux/4 -> [Vs]
  Demux/3 -> [Qs]
  Demux/2 -> [ws]
  Demux/1 -> [Ps]
  [wt] -> Mux5/5
  [V] -> Mux5/4
  [Q] -> Mux5/3
  [f] -> Gain/1
  Mux5/1 -> [m]
  [P] -> Mux5/1
  [w] -> Mux5/2
  [Qs] -> Gain3/1
  [Ps] -> Gain5/1
  [vodq] -> GFL Current Loop/3
  [isdq] -> GFL Current Loop/2
  [Isdq_ref] -> GFL Current Loop/1
  GFL Current Loop/1 -> [Uref]
  B1/1 -> Memory/1
  [wt] -> abc to dq3/2
  Selector3/1 -> [vodq]
  [vo] -> abc to dq3/1
  abc to dq3/1 -> Selector3/1
  [wt] -> abc to dq4/2
  abc to dq4/1 -> Selector6/1
  Selector6/1 -> [isdq]
  [wt] -> GFL Current Loop/4
  B2/2 -> Memory2/1
  B1/2 -> Memory1/1
  "GFL Droop "/1 -> [PQref]
  GFL Power Loop/1 -> [Isdq_ref]
  u/1 -> Bus Selector/1
  [Ps] -> "GFL Droop "/3
  [Vs] -> "GFL Droop "/4
  [ws] -> "GFL Droop "/1
  [Qs] -> "GFL Droop "/6
  Gain/1 -> "GFL Droop "/2
  [V] -> "GFL Droop "/5
  [PQref] -> GFL Power Loop/1
  [PQ] -> GFL Power Loop/2
  Mux/1 -> [fig]
  [f] -> Mux/1
  [P] -> Gain7/1
  [V] -> Gain4/1
  [vodq] -> Square/1
  Sum of Elements/1 -> Sqrt2/1
  [Q] -> Gain2/1
  Memory2/1 -> [is]
  Memory/1 -> [vo]
  Memory1/1 -> [io]
  [is] -> abc to dq4/1
  Memory3/1 -> [vs]
  B2/1 -> Memory3/1
  [vo] -> PLL/1
  PLL/2 -> [wt]
  PLL/1 -> [f]
  Bus Creator/1 -> m/1
  [droop] -> Bus Creator/2  "droop"
  [iloop] -> Bus Creator/3  "current"
  [vloop] -> Bus Creator/4  "voltage"
  [fig] -> Bus Creator/1  "fig"
  PLL/3 -> [w]
  [w] -> GFL Current Loop/5
  [vs] -> Mux1/1
  [is] -> Mux1/2
  [vo] -> Mux1/3
  [io] -> Mux1/4
  Mux1/1 -> [vi]
  [vs] -> abc to dq5/1
  Selector1/1 -> [vsdq]
  [wt] -> abc to dq5/2
  abc to dq5/1 -> Selector1/1
  [vsdq] -> Mux2/1
  [isdq] -> Mux2/2
  [vodq] -> Mux2/3
  Mux2/1 -> [vidq]
  [vidq] -> Bus Creator/5  "vidq"
  [vi] -> Bus Creator/6  "vi"
  [m] -> Bus Creator/7  "m"
  [io] -> abc to dq6/1
  abc to dq6/1 -> Selector4/1
  [wt] -> abc to dq6/2
  Selector4/1 -> [iodq]
  [iodq] -> Mux2/4
  Square/1 -> Sum of Elements/1
  [isdq] -> Power calculation/2
  [vodq] -> Power calculation/1
  [Uref] -> Universal Bridge/1
  Power calculation/1 -> Demux1/1, [PQ]
  Demux1/1 -> [P]
  Demux1/2 -> [Q]
  Sqrt2/1 -> [V]
  Gain7/1 -> Mux/2
  Gain5/1 -> Mux/3
  Bus Selector/1 -> [refs]  "<refs>"
  [iodq] -> Mux4/2
  Mux4/1 -> Gain1/1
  Selector/1 -> Mux/4
  Gain4/1 -> Mux/5
  Gain2/1 -> Mux/6
  Gain3/1 -> Mux/7
  Selector2/1 -> Mux/8
  Gain1/1 -> Selector2/1, Selector/1
  Bus Selector/2 -> Demux/1  "<us>"
  connections:
  Universal Bridge/RConn2 -- DC Voltage Source1/LConn1
  Universal Bridge/RConn1 -- DC Voltage Source1/RConn1
  RL_c2/LConn1 -- B1/LConn3
  B2/LConn2 -- Universal Bridge/LConn2
  B2/LConn1 -- Universal Bridge/LConn1
  B2/LConn3 -- Universal Bridge/LConn3
  C/RConn1 -- B1/RConn3
  B1/RConn2 -- B/RConn1
  B1/RConn1 -- A/RConn1
  B1/LConn1 -- RL_c/LConn1
  RL_c1/LConn1 -- B1/LConn2
  RL_c2/RConn1 -- B2/RConn3
  RL_c1/RConn1 -- B2/RConn2
  B2/RConn1 -- RL_c/RConn1

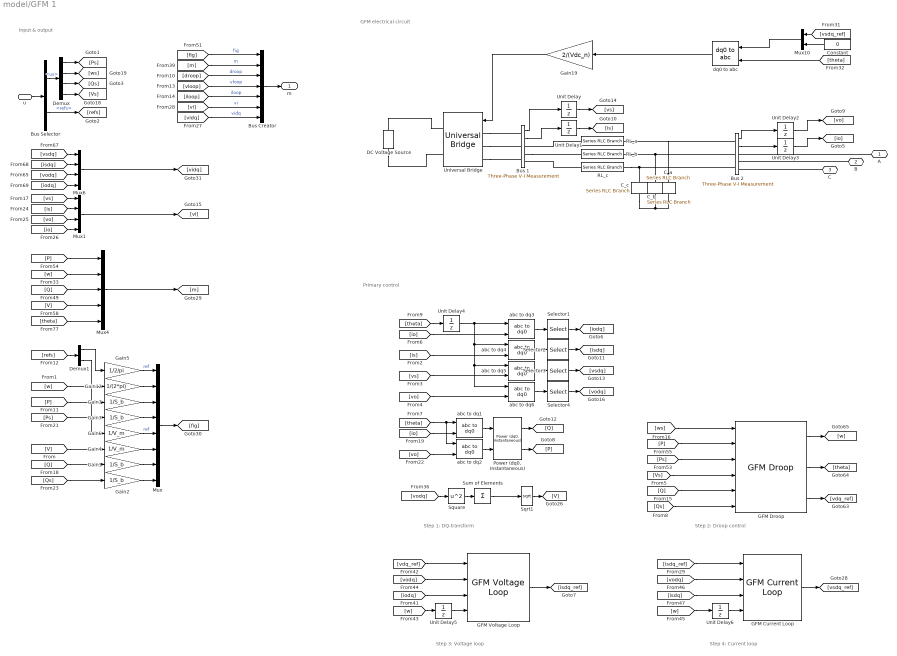
== system model/GFM 1 ==
  note: Primary control
  note: Input & output
  note: Step 4: Current loop
  note: Step 3: Voltage loop
  note: Step 2: Droop control
  note: Step 1: DQ-transform
  note: GFM electrical circuit
  u : Inport
  Bus Creator : BusCreator  Inputs=7
  Bus Selector : BusSelector  OutputSignals=us,refs
  Bus 1 : spsThreePhaseVIMeasurementLib/Three-Phase V-I Measurement  VoltageMeasurement=phase-to-ground  SetLabelV=off  LabelV=is  Vpu=off  VpuLL=off  CurrentMeasurement=yes  SetLabelI=off  LabelI=Iabc_5  Ipu=off  Pbase=S_b  Vbase=V_b  OutputType=Complex  PhasorSimulation=off  PSBequivalent=0
  Bus 2 : spsThreePhaseVIMeasurementLib/Three-Phase V-I Measurement  VoltageMeasurement=phase-to-ground  SetLabelV=off  LabelV=is  Vpu=off  VpuLL=off  CurrentMeasurement=yes  SetLabelI=off  LabelI=Iabc_5  Ipu=off  Pbase=S_b  Vbase=V_b  OutputType=Complex  PhasorSimulation=off  PSBequivalent=0
  C_a : spsSeriesRLCBranchLib/Series RLC Branch  LConnTagsString=__new0  RConnTagsString=__new0  BranchType=C  Resistance=1  Inductance=1e-3  SetiL0=off  InitialCurrent=0  Capacitance=pIBR.RLC(3)  Setx0=off  InitialVoltage=165  Measurements=Branch voltage and current
  C_b : spsSeriesRLCBranchLib/Series RLC Branch  LConnTagsString=__new0  RConnTagsString=__new0  BranchType=C  Resistance=1  Inductance=1e-3  SetiL0=off  InitialCurrent=0  Capacitance=pIBR.RLC(3)  Setx0=off  InitialVoltage=165  Measurements=Branch voltage and current
  C_c : spsSeriesRLCBranchLib/Series RLC Branch  LConnTagsString=__new0  RConnTagsString=__new0  BranchType=C  Resistance=1  Inductance=1e-3  SetiL0=off  InitialCurrent=0  Capacitance=pIBR.RLC(3)  Setx0=off  InitialVoltage=165  Measurements=Branch voltage and current
  Constant : Constant  Value=0
  DC Voltage Source : spsDCVoltageSourceLib/DC Voltage Source  Amplitude=Vdc_n  Measurements=None
  Demux : Demux
  Demux1 : Demux  Outputs=2
  GFM Current Loop : lib_IBR/GFM Current Loop  SystemSampleTime=-1  VariantActivationTime=update diagram  AllowFlexibleInterface=on  Latency=0  AutoFrameSizeCalculation=off
  GFM Droop : lib_IBR/GFM Droop  SystemSampleTime=-1  VariantActivationTime=update diagram  AllowFlexibleInterface=on  Latency=0  AutoFrameSizeCalculation=off
  GFM Voltage Loop : lib_IBR/GFM Voltage Loop  SystemSampleTime=-1  VariantActivationTime=update diagram  AllowFlexibleInterface=on  Latency=0  AutoFrameSizeCalculation=off
  Gain{1..3,7} (4 alike) : Gain  Gain=1/S_b
  Gain12 : Gain  Gain=1/(2*pi)
  Gain19 : Gain  Gain=2/(Vdc_n)
  Gain4 : Gain  Gain=1/V_m
  Gain5 : Gain  Gain=1/2/pi
  Gain6 : Gain  Gain=1/V_m
  Mux : Mux  Inputs=8
  Mux1 : Mux
  Mux10 : Mux  Inputs=2
  Mux4 : Mux  Inputs=5
  Mux6 : Mux
  "Power (dq0, Instantaneous)" : spsPowerdq0InstantaneousLib/Power (dq0, Instantaneous)
      settings: LibrarySourceBlock=|
      | sps_lib/Sensors and Measurements/Power
      | (dq0, Instantaneous)
  RL_a : spsSeriesRLCBranchLib/Series RLC Branch  LConnTagsString=__new0  RConnTagsString=__new0  BranchType=RL  Resistance=pIBR.RLC(1)  Inductance=pIBR.RLC(2)  SetiL0=off  InitialCurrent=0  Capacitance=1e-6  Setx0=off  InitialVoltage=0  Measurements=Branch voltage and current
  RL_b : spsSeriesRLCBranchLib/Series RLC Branch  LConnTagsString=__new0  RConnTagsString=__new0  BranchType=RL  Resistance=pIBR.RLC(1)  Inductance=pIBR.RLC(2)  SetiL0=off  InitialCurrent=0  Capacitance=1e-6  Setx0=off  InitialVoltage=0  Measurements=Branch voltage and current
  RL_c : spsSeriesRLCBranchLib/Series RLC Branch  LConnTagsString=__new0  RConnTagsString=__new0  BranchType=RL  Resistance=pIBR.RLC(1)  Inductance=pIBR.RLC(2)  SetiL0=off  InitialCurrent=0  Capacitance=1e-6  Setx0=off  InitialVoltage=0  Measurements=Branch voltage and current
  Selector{1..4} (4 alike) : Selector  InputPortWidth=3  IndexOptions=Index vector (dialog)  Indices=[1 2]  OutputSizes=1
  Sqrt1 : Sqrt
  Square : Math  Operator=square
  Sum of Elements : Sum  Inputs=+
  Unit Delay{,1..6} (7 alike) : UnitDelay  SampleTime=Ts  HasFrameUpgradeWarning=on
  Universal Bridge : spsUniversalBridgeLib/Universal Bridge  Arms=3  SnubberResistance=1e5  SnubberCapacitance=inf  Device=Average-model based VSC  Ron=1e-3  Lon=0  ForwardVoltages="[  0  0  ]"  ForwardVoltage=0  GTOparameters=[ 10e-6 , 20e-6 ]  IGBTparameters=[ 1e-6 , 2e-6 ]  Measurements=All voltages and currents  Measurements_2=Voltages and Currents  converterType=Rectifier
  abc to dq{1..6} (6 alike) : spsabctodq0Lib/abc to dq0  Alignment=90 degrees behind phase A axis
  dq0 to abc : spsdq0toabcLib/dq0 to abc  Alignment=90 degrees behind phase A axis
  A : PMIOPort  Side=Right
  B : PMIOPort  Port=2  Side=Right
  C : PMIOPort  Port=3  Side=Right
  m : Outport  VectorParamsAs1DForOutWhenUnconnected=off
  wires:
  Demux/4 -> [Vs]
  Demux/3 -> [Qs]
  Demux/2 -> [ws]
  Demux/1 -> [Ps]
  [theta] -> Mux4/5
  [V] -> Mux4/4
  [Q] -> Mux4/3
  [w] -> Mux4/2
  [P] -> Mux4/1
  Gain6/1 -> Mux/5  "ref"
  Demux1/2 -> Gain6/1
  Demux1/1 -> Gain5/1
  Gain5/1 -> Mux/1  "ref"
  Gain4/1 -> Mux/6
  Gain1/1 -> Mux/7
  Gain3/1 -> Mux/4
  [ws] -> GFM Droop/1
  [Ps] -> GFM Droop/3
  [Vs] -> GFM Droop/4
  [P] -> GFM Droop/2
  GFM Droop/1 -> [w]
  GFM Droop/3 -> [vdq_ref]
  [Q] -> GFM Droop/5
  [Qs] -> GFM Droop/6
  GFM Droop/2 -> [theta]
  Unit Delay1/1 -> [is]
  Unit Delay6/1 -> GFM Current Loop/4
  Unit Delay5/1 -> GFM Voltage Loop/4
  [droop] -> Bus Creator/3  "droop"
  [w] -> Unit Delay6/1
  [w] -> Unit Delay5/1
  [vidq] -> Bus Creator/7  "vidq"
  [vi] -> Bus Creator/6  "vi"
  Mux1/1 -> [vi]
  [iloop] -> Bus Creator/5  "iloop"
  [vloop] -> Bus Creator/4  "vloop"
  Mux10/1 -> dq0 to abc/1
  [vsdq_ref] -> Mux10/1
  Constant/1 -> Mux10/2
  Square/1 -> Sum of Elements/1
  [vodq] -> Square/1
  Selector2/1 -> [isdq]
  Selector3/1 -> [vsdq]
  Selector4/1 -> [vodq]
  Selector1/1 -> [iodq]
  Mux6/1 -> [vidq]
  [theta] -> Unit Delay4/1
  Unit Delay4/1 -> abc to dq3/2, abc to dq4/2, abc to dq5/2, abc to dq6/2
  Bus 1/1 -> Unit Delay/1
  [fig] -> Bus Creator/1  "fig"
  Mux/1 -> [fig]
  [m] -> Bus Creator/2  "m"
  Bus Creator/1 -> m/1
  Mux4/1 -> [m]
  Sum of Elements/1 -> Sqrt1/1
  Sqrt1/1 -> [V]
  [isdq_ref] -> GFM Current Loop/1
  GFM Voltage Loop/1 -> [isdq_ref]
  Gain7/1 -> Mux/3
  [P] -> Gain7/1
  [V] -> Gain4/1
  Gain12/1 -> Mux/2
  [w] -> Gain12/1
  abc to dq1/1 -> "Power (dq0, Instantaneous)"/2
  abc to dq2/1 -> "Power (dq0, Instantaneous)"/1
  [theta] -> abc to dq2/2, abc to dq1/2
  [vo] -> abc to dq2/1
  "Power (dq0, Instantaneous)"/2 -> [Q]
  "Power (dq0, Instantaneous)"/1 -> [P]
  [io] -> abc to dq1/1
  [io] -> abc to dq3/1
  [is] -> abc to dq4/1
  [vo] -> abc to dq6/1
  [vs] -> abc to dq5/1
  abc to dq3/1 -> Selector1/1
  abc to dq4/1 -> Selector2/1
  abc to dq5/1 -> Selector3/1
  abc to dq6/1 -> Selector4/1
  [theta] -> dq0 to abc/2
  dq0 to abc/1 -> Gain19/1
  [vdq_ref] -> GFM Voltage Loop/1
  [iodq] -> GFM Voltage Loop/3
  [vodq] -> GFM Current Loop/2
  [isdq] -> GFM Current Loop/3
  GFM Current Loop/1 -> [vsdq_ref]
  [vodq] -> GFM Voltage Loop/2
  Gain19/1 -> Universal Bridge/1
  Unit Delay3/1 -> [io]
  Bus 2/2 -> Unit Delay3/1
  Unit Delay2/1 -> [vo]
  Bus 2/1 -> Unit Delay2/1
  Bus 1/2 -> Unit Delay1/1
  Unit Delay/1 -> [vs]
  [Q] -> Gain1/1
  [Ps] -> Gain3/1
  [Qs] -> Gain2/1
  Gain2/1 -> Mux/8
  [vodq] -> Mux6/3
  [iodq] -> Mux6/4
  [isdq] -> Mux6/2
  [vsdq] -> Mux6/1
  [io] -> Mux1/4
  [vo] -> Mux1/3
  [is] -> Mux1/2
  [vs] -> Mux1/1
  u/1 -> Bus Selector/1
  Bus Selector/1 -> Demux/1  "<us>"
  Bus Selector/2 -> [refs]  "<refs>"
  [refs] -> Demux1/1
  connections:
  RL_c/LConn1 -- Bus 1/RConn3
  RL_a/LConn1 -- Bus 1/RConn1
  Bus 2/LConn2 -- RL_b/RConn1 -- C_b/LConn1
  RL_c/RConn1 -- Bus 2/LConn3 -- C_c/LConn1
  Bus 1/RConn2 -- RL_b/LConn1
  DC Voltage Source/RConn1 -- Universal Bridge/RConn1
  C/RConn1 -- Bus 2/RConn3
  B/RConn1 -- Bus 2/RConn2
  A/RConn1 -- Bus 2/RConn1
  Universal Bridge/LConn3 -- Bus 1/LConn3
  Universal Bridge/LConn2 -- Bus 1/LConn2
  Universal Bridge/LConn1 -- Bus 1/LConn1
  DC Voltage Source/LConn1 -- Universal Bridge/RConn2
  C_c/RConn1 -- C_b/RConn1 -- C_a/RConn1
  C_a/LConn1 -- RL_a/RConn1 -- Bus 2/LConn1

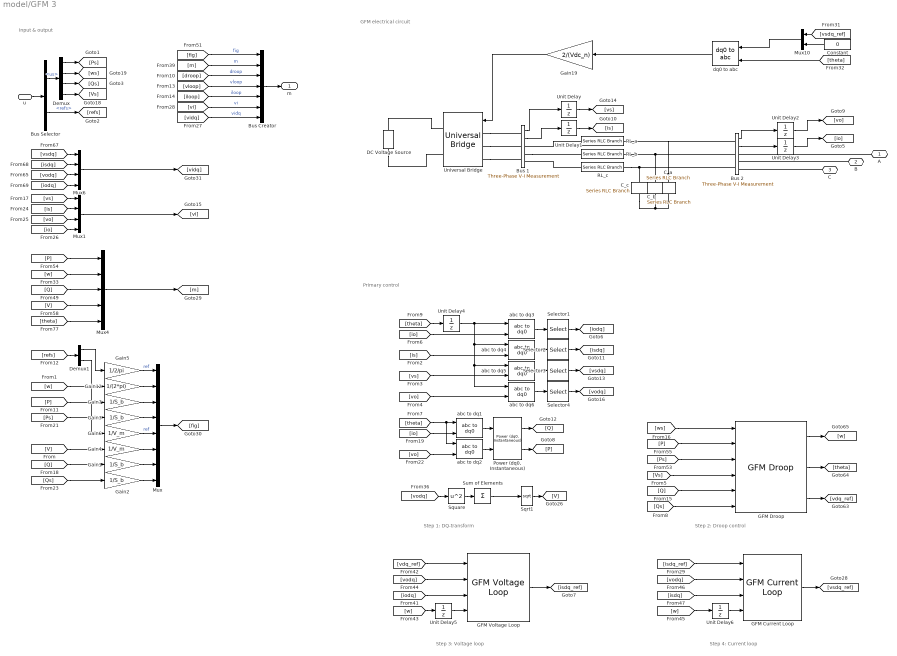
== system model/GFM 3 ==
  note: Primary control
  note: Input & output
  note: Step 4: Current loop
  note: Step 3: Voltage loop
  note: Step 2: Droop control
  note: Step 1: DQ-transform
  note: GFM electrical circuit
  u : Inport
  Bus Creator : BusCreator  Inputs=7
  Bus Selector : BusSelector  OutputSignals=us,refs
  Bus 1 : spsThreePhaseVIMeasurementLib/Three-Phase V-I Measurement  VoltageMeasurement=phase-to-ground  SetLabelV=off  LabelV=is  Vpu=off  VpuLL=off  CurrentMeasurement=yes  SetLabelI=off  LabelI=Iabc_5  Ipu=off  Pbase=S_b  Vbase=V_b  OutputType=Complex  PhasorSimulation=off  PSBequivalent=0
  Bus 2 : spsThreePhaseVIMeasurementLib/Three-Phase V-I Measurement  VoltageMeasurement=phase-to-ground  SetLabelV=off  LabelV=is  Vpu=off  VpuLL=off  CurrentMeasurement=yes  SetLabelI=off  LabelI=Iabc_5  Ipu=off  Pbase=S_b  Vbase=V_b  OutputType=Complex  PhasorSimulation=off  PSBequivalent=0
  C_a : spsSeriesRLCBranchLib/Series RLC Branch  LConnTagsString=__new0  RConnTagsString=__new0  BranchType=C  Resistance=1  Inductance=1e-3  SetiL0=off  InitialCurrent=0  Capacitance=pIBR.RLC(3)  Setx0=off  InitialVoltage=165  Measurements=Branch voltage and current
  C_b : spsSeriesRLCBranchLib/Series RLC Branch  LConnTagsString=__new0  RConnTagsString=__new0  BranchType=C  Resistance=1  Inductance=1e-3  SetiL0=off  InitialCurrent=0  Capacitance=pIBR.RLC(3)  Setx0=off  InitialVoltage=165  Measurements=Branch voltage and current
  C_c : spsSeriesRLCBranchLib/Series RLC Branch  LConnTagsString=__new0  RConnTagsString=__new0  BranchType=C  Resistance=1  Inductance=1e-3  SetiL0=off  InitialCurrent=0  Capacitance=pIBR.RLC(3)  Setx0=off  InitialVoltage=165  Measurements=Branch voltage and current
  Constant : Constant  Value=0
  DC Voltage Source : spsDCVoltageSourceLib/DC Voltage Source  Amplitude=Vdc_n  Measurements=None
  Demux : Demux
  Demux1 : Demux  Outputs=2
  GFM Current Loop : lib_IBR/GFM Current Loop  SystemSampleTime=-1  VariantActivationTime=update diagram  AllowFlexibleInterface=on  Latency=0  AutoFrameSizeCalculation=off
  GFM Droop : lib_IBR/GFM Droop  SystemSampleTime=-1  VariantActivationTime=update diagram  AllowFlexibleInterface=on  Latency=0  AutoFrameSizeCalculation=off
  GFM Voltage Loop : lib_IBR/GFM Voltage Loop  SystemSampleTime=-1  VariantActivationTime=update diagram  AllowFlexibleInterface=on  Latency=0  AutoFrameSizeCalculation=off
  Gain{1..3,7} (4 alike) : Gain  Gain=1/S_b
  Gain12 : Gain  Gain=1/(2*pi)
  Gain19 : Gain  Gain=2/(Vdc_n)
  Gain4 : Gain  Gain=1/V_m
  Gain5 : Gain  Gain=1/2/pi
  Gain6 : Gain  Gain=1/V_m
  Mux : Mux  Inputs=8
  Mux1 : Mux
  Mux10 : Mux  Inputs=2
  Mux4 : Mux  Inputs=5
  Mux6 : Mux
  "Power (dq0, Instantaneous)" : spsPowerdq0InstantaneousLib/Power (dq0, Instantaneous)
      settings: LibrarySourceBlock=|
      | sps_lib/Sensors and Measurements/Power
      | (dq0, Instantaneous)
  RL_a : spsSeriesRLCBranchLib/Series RLC Branch  LConnTagsString=__new0  RConnTagsString=__new0  BranchType=RL  Resistance=pIBR.RLC(1)  Inductance=pIBR.RLC(2)  SetiL0=off  InitialCurrent=0  Capacitance=1e-6  Setx0=off  InitialVoltage=0  Measurements=Branch voltage and current
  RL_b : spsSeriesRLCBranchLib/Series RLC Branch  LConnTagsString=__new0  RConnTagsString=__new0  BranchType=RL  Resistance=pIBR.RLC(1)  Inductance=pIBR.RLC(2)  SetiL0=off  InitialCurrent=0  Capacitance=1e-6  Setx0=off  InitialVoltage=0  Measurements=Branch voltage and current
  RL_c : spsSeriesRLCBranchLib/Series RLC Branch  LConnTagsString=__new0  RConnTagsString=__new0  BranchType=RL  Resistance=pIBR.RLC(1)  Inductance=pIBR.RLC(2)  SetiL0=off  InitialCurrent=0  Capacitance=1e-6  Setx0=off  InitialVoltage=0  Measurements=Branch voltage and current
  Selector{1..4} (4 alike) : Selector  InputPortWidth=3  IndexOptions=Index vector (dialog)  Indices=[1 2]  OutputSizes=1
  Sqrt1 : Sqrt
  Square : Math  Operator=square
  Sum of Elements : Sum  Inputs=+
  Unit Delay{,1..6} (7 alike) : UnitDelay  SampleTime=Ts  HasFrameUpgradeWarning=on
  Universal Bridge : spsUniversalBridgeLib/Universal Bridge  Arms=3  SnubberResistance=1e5  SnubberCapacitance=inf  Device=Average-model based VSC  Ron=1e-3  Lon=0  ForwardVoltages="[  0  0  ]"  ForwardVoltage=0  GTOparameters=[ 10e-6 , 20e-6 ]  IGBTparameters=[ 1e-6 , 2e-6 ]  Measurements=All voltages and currents  Measurements_2=Voltages and Currents  converterType=Rectifier
  abc to dq{1..6} (6 alike) : spsabctodq0Lib/abc to dq0  Alignment=90 degrees behind phase A axis
  dq0 to abc : spsdq0toabcLib/dq0 to abc  Alignment=90 degrees behind phase A axis
  A : PMIOPort  Side=Right
  B : PMIOPort  Port=2  Side=Right
  C : PMIOPort  Port=3  Side=Right
  m : Outport  VectorParamsAs1DForOutWhenUnconnected=off
  wires:
  Demux/4 -> [Vs]
  Demux/3 -> [Qs]
  Demux/2 -> [ws]
  Demux/1 -> [Ps]
  [theta] -> Mux4/5
  [V] -> Mux4/4
  [Q] -> Mux4/3
  [w] -> Mux4/2
  [P] -> Mux4/1
  Gain6/1 -> Mux/5  "ref"
  Demux1/2 -> Gain6/1
  Demux1/1 -> Gain5/1
  Gain5/1 -> Mux/1  "ref"
  Gain4/1 -> Mux/6
  Gain1/1 -> Mux/7
  Gain3/1 -> Mux/4
  [ws] -> GFM Droop/1
  [Ps] -> GFM Droop/3
  [Vs] -> GFM Droop/4
  [P] -> GFM Droop/2
  GFM Droop/1 -> [w]
  GFM Droop/3 -> [vdq_ref]
  [Q] -> GFM Droop/5
  [Qs] -> GFM Droop/6
  GFM Droop/2 -> [theta]
  Unit Delay1/1 -> [is]
  Unit Delay6/1 -> GFM Current Loop/4
  Unit Delay5/1 -> GFM Voltage Loop/4
  [droop] -> Bus Creator/3  "droop"
  [w] -> Unit Delay6/1
  [w] -> Unit Delay5/1
  [vidq] -> Bus Creator/7  "vidq"
  [vi] -> Bus Creator/6  "vi"
  Mux1/1 -> [vi]
  [iloop] -> Bus Creator/5  "iloop"
  [vloop] -> Bus Creator/4  "vloop"
  Mux10/1 -> dq0 to abc/1
  [vsdq_ref] -> Mux10/1
  Constant/1 -> Mux10/2
  Square/1 -> Sum of Elements/1
  [vodq] -> Square/1
  Selector2/1 -> [isdq]
  Selector3/1 -> [vsdq]
  Selector4/1 -> [vodq]
  Selector1/1 -> [iodq]
  Mux6/1 -> [vidq]
  [theta] -> Unit Delay4/1
  Unit Delay4/1 -> abc to dq3/2, abc to dq4/2, abc to dq5/2, abc to dq6/2
  Bus 1/1 -> Unit Delay/1
  [fig] -> Bus Creator/1  "fig"
  Mux/1 -> [fig]
  [m] -> Bus Creator/2  "m"
  Bus Creator/1 -> m/1
  Mux4/1 -> [m]
  Sum of Elements/1 -> Sqrt1/1
  Sqrt1/1 -> [V]
  [isdq_ref] -> GFM Current Loop/1
  GFM Voltage Loop/1 -> [isdq_ref]
  Gain7/1 -> Mux/3
  [P] -> Gain7/1
  [V] -> Gain4/1
  Gain12/1 -> Mux/2
  [w] -> Gain12/1
  abc to dq1/1 -> "Power (dq0, Instantaneous)"/2
  abc to dq2/1 -> "Power (dq0, Instantaneous)"/1
  [theta] -> abc to dq2/2, abc to dq1/2
  [vo] -> abc to dq2/1
  "Power (dq0, Instantaneous)"/2 -> [Q]
  "Power (dq0, Instantaneous)"/1 -> [P]
  [io] -> abc to dq1/1
  [io] -> abc to dq3/1
  [is] -> abc to dq4/1
  [vo] -> abc to dq6/1
  [vs] -> abc to dq5/1
  abc to dq3/1 -> Selector1/1
  abc to dq4/1 -> Selector2/1
  abc to dq5/1 -> Selector3/1
  abc to dq6/1 -> Selector4/1
  [theta] -> dq0 to abc/2
  dq0 to abc/1 -> Gain19/1
  [vdq_ref] -> GFM Voltage Loop/1
  [iodq] -> GFM Voltage Loop/3
  [vodq] -> GFM Current Loop/2
  [isdq] -> GFM Current Loop/3
  GFM Current Loop/1 -> [vsdq_ref]
  [vodq] -> GFM Voltage Loop/2
  Gain19/1 -> Universal Bridge/1
  Unit Delay3/1 -> [io]
  Bus 2/2 -> Unit Delay3/1
  Unit Delay2/1 -> [vo]
  Bus 2/1 -> Unit Delay2/1
  Bus 1/2 -> Unit Delay1/1
  Unit Delay/1 -> [vs]
  [Q] -> Gain1/1
  [Ps] -> Gain3/1
  [Qs] -> Gain2/1
  Gain2/1 -> Mux/8
  [vodq] -> Mux6/3
  [iodq] -> Mux6/4
  [isdq] -> Mux6/2
  [vsdq] -> Mux6/1
  [io] -> Mux1/4
  [vo] -> Mux1/3
  [is] -> Mux1/2
  [vs] -> Mux1/1
  u/1 -> Bus Selector/1
  Bus Selector/1 -> Demux/1  "<us>"
  Bus Selector/2 -> [refs]  "<refs>"
  [refs] -> Demux1/1
  connections:
  RL_c/LConn1 -- Bus 1/RConn3
  RL_a/LConn1 -- Bus 1/RConn1
  Bus 2/LConn2 -- RL_b/RConn1 -- C_b/LConn1
  RL_c/RConn1 -- Bus 2/LConn3 -- C_c/LConn1
  Bus 1/RConn2 -- RL_b/LConn1
  DC Voltage Source/RConn1 -- Universal Bridge/RConn1
  C/RConn1 -- Bus 2/RConn3
  B/RConn1 -- Bus 2/RConn2
  A/RConn1 -- Bus 2/RConn1
  Universal Bridge/LConn3 -- Bus 1/LConn3
  Universal Bridge/LConn2 -- Bus 1/LConn2
  Universal Bridge/LConn1 -- Bus 1/LConn1
  DC Voltage Source/LConn1 -- Universal Bridge/RConn2
  C_c/RConn1 -- C_b/RConn1 -- C_a/RConn1
  C_a/LConn1 -- RL_a/RConn1 -- Bus 2/LConn1

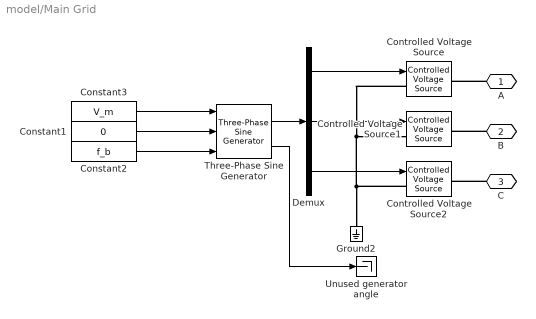
== system model/Main Grid ==
  Constant1 : Constant  Value=0
  Constant2 : Constant  Value=f_b
  Constant3 : Constant  Value=V_m
  Controlled Voltage Source : spsControlledVoltageSourceLib/Controlled Voltage Source  Initialize=on  Source_Type=AC  Amplitude=0  Phase=0  Frequency=0  Measurements=None
  Controlled Voltage Source1 : spsControlledVoltageSourceLib/Controlled Voltage Source  Initialize=on  Source_Type=AC  Amplitude=0  Phase=0  Frequency=0  Measurements=None
  Controlled Voltage Source2 : spsControlledVoltageSourceLib/Controlled Voltage Source  Initialize=on  Source_Type=AC  Amplitude=0  Phase=0  Frequency=0  Measurements=None
  Demux : Demux  Outputs=3
  Ground2 : spsGroundLib/Ground  LConnTagsString=a
  Three-Phase Sine Generator : spsThreePhaseSineGeneratorLib/Three-Phase Sine Generator  Ts=Ts
      settings: LibrarySourceBlock=|
      | sps_lib/Sources/Signal Generator Sources/Three-Phase
      | Sine Generator
  Unused generator angle : Terminator
  A : PMIOPort  Side=Right
  B : PMIOPort  Port=2  Side=Right
  C : PMIOPort  Port=3  Side=Right
  wires:
  Three-Phase Sine Generator/1 -> Demux/1
  Demux/1 -> Controlled Voltage Source/1
  Demux/2 -> Controlled Voltage Source1/1
  Demux/3 -> Controlled Voltage Source2/1
  Constant2/1 -> Three-Phase Sine Generator/3
  Constant3/1 -> Three-Phase Sine Generator/1
  Constant1/1 -> Three-Phase Sine Generator/2
  Three-Phase Sine Generator/2 -> Unused generator angle/1
  connections:
  A/RConn1 -- Controlled Voltage Source/RConn1
  B/RConn1 -- Controlled Voltage Source1/RConn1
  C/RConn1 -- Controlled Voltage Source2/RConn1
  Controlled Voltage Source2/LConn1 -- Controlled Voltage Source/LConn1 -- Controlled Voltage Source1/LConn1 -- Ground2/LConn1

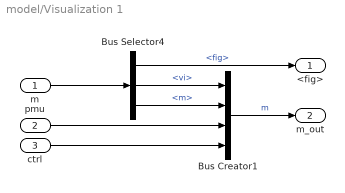
== system model/Visualization 1 ==
  m : Inport
  pmu : Inport  Port=2
  ctrl : Inport  Port=3
  Bus Creator1 : BusCreator  Inputs=4
  Bus Selector4 : BusSelector  OutputSignals=fig,vi,m
  <fig> : Outport
  m_out : Outport  Port=2
  wires:
  Bus Creator1/1 -> m_out/1  "m"
  Bus Selector4/2 -> Bus Creator1/1  "<vi>"
  Bus Selector4/1 -> <fig>/1  "<fig>"
  Bus Selector4/3 -> Bus Creator1/2  "<m>"
  pmu/1 -> Bus Creator1/3
  m/1 -> Bus Selector4/1
  ctrl/1 -> Bus Creator1/4

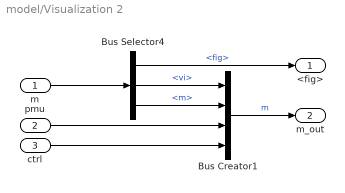
== system model/Visualization 2 ==
  m : Inport
  pmu : Inport  Port=2
  ctrl : Inport  Port=3
  Bus Creator1 : BusCreator  Inputs=4
  Bus Selector4 : BusSelector  OutputSignals=fig,vi,m
  <fig> : Outport
  m_out : Outport  Port=2
  wires:
  ctrl/1 -> Bus Creator1/4
  m/1 -> Bus Selector4/1
  pmu/1 -> Bus Creator1/3
  Bus Selector4/3 -> Bus Creator1/2  "<m>"
  Bus Selector4/1 -> <fig>/1  "<fig>"
  Bus Selector4/2 -> Bus Creator1/1  "<vi>"
  Bus Creator1/1 -> m_out/1  "m"

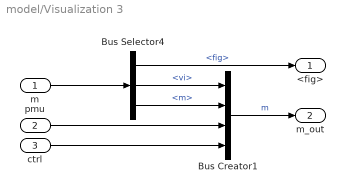
== system model/Visualization 3 ==
  m : Inport
  pmu : Inport  Port=2
  ctrl : Inport  Port=3
  Bus Creator1 : BusCreator  Inputs=4
  Bus Selector4 : BusSelector  OutputSignals=fig,vi,m
  <fig> : Outport
  m_out : Outport  Port=2
  wires:
  Bus Creator1/1 -> m_out/1  "m"
  Bus Selector4/2 -> Bus Creator1/1  "<vi>"
  Bus Selector4/1 -> <fig>/1  "<fig>"
  Bus Selector4/3 -> Bus Creator1/2  "<m>"
  pmu/1 -> Bus Creator1/3
  m/1 -> Bus Selector4/1
  ctrl/1 -> Bus Creator1/4

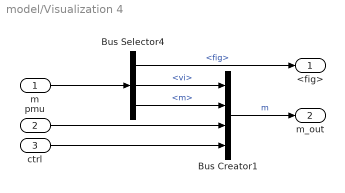
== system model/Visualization 4 ==
  m : Inport
  pmu : Inport  Port=2
  ctrl : Inport  Port=3
  Bus Creator1 : BusCreator  Inputs=4
  Bus Selector4 : BusSelector  OutputSignals=fig,vi,m
  <fig> : Outport
  m_out : Outport  Port=2
  wires:
  ctrl/1 -> Bus Creator1/4
  m/1 -> Bus Selector4/1
  pmu/1 -> Bus Creator1/3
  Bus Selector4/3 -> Bus Creator1/2  "<m>"
  Bus Selector4/1 -> <fig>/1  "<fig>"
  Bus Selector4/2 -> Bus Creator1/1  "<vi>"
  Bus Creator1/1 -> m_out/1  "m"
